simulink model "afe_inv_psm_n"  (R2026b)
settings: Solver=ode23tb  StopTime=param.sim.simlength  FixedStep=param.sim.tc  MaxStep=param.glb_time.tc
values from neighbouring files (symbols this model uses):
  param = struct()    [init_model.m]
libraries: fl_lib x30, nesl_utility x17, single_phase_transformer_lib x3, grid_following_dqctrl x2, pmsm_inverter_dqctrl x2, cstblocks_lti x2, three_phase_voltage_with_frt_emulator_mfcn x1, simple_flexible_shaft x1, permanent_magnet_synchronous_machine x1
(part 1 of 2)
settings Model: Creator=dbagn  LastModifiedBy=d.bagnara
settings SolverCC: SolverResetMethod=Robust  ZeroCrossControl=DisableAll
settings DataIOCC: DSMLogging=off  ReturnWorkspaceOutputs=off  SaveOutput=off  SaveTime=off  SignalLogging=off
settings OptimizationCC: ReuseModelBlockBuffer=off
settings SFSimCC: CustomCodeUndefinedFunction=ThrowError  DefaultCustomCodeDeterministicFunctions=All
settings SFSimCC: SimCustomHeaderCode=|
  | #include "rpi.h"
  | #include "mavgflt.h"
  | #include "mavgflt_simulink.h"
  | #include "mavgflts.h"
  | #include "mavgflts_simulink.h"
  | #include "dsmavgflt.h"
  | #include "dsmavgflt_simulink.h"
  | #include "bemf_obsv.h"
  | #include "bemf_obsv_simulink.h"
  | #include "bemf_obsv_load_est.h"
  | #include "bemf_obsv_load_est_simulink.h"
  | #include "dqvector_pi.h"
  | #include "dqvector_pi_simulink.h"
  | #include "sv_pwm_simulink.h"
  | #include "sv_pwm.h"
  | #include "first_harmonic_tracker.h"
  | #include "first_harmonic_tracker_simulink.h"
  | #include "dqpll_thyr.h"
  | #include "dqpll_thyr_simulink.h"
  | #include "dqpll_grid.h"
  | #include "dqpll_grid_simulink.h"
  | #include "linear_double_integrator_observer_simulink.h"
  | #include "linear_double_integrator_observer.h"
  | #include "sv_pwm_cm_simulink.h"
  | #include "sv_pwm_cm.h"
settings SFSimCC: SimUserIncludeDirs=|
  | include
  | src
settings SFSimCC: SimUserSources=|
  | "rpi.c"
  | "mavgflt_simulink.c"
  | "mavgflt.c"
  | "mavgflts_simulink.c"
  | "mavgflts.c"
  | "dsmavgflt_simulink.c"
  | "dsmavgflt.c"
  | "bemf_obsv_simulink.c"
  | "bemf_obsv.c"
  | "bemf_obsv_load_est_simulink.c"
  | "bemf_obsv_load_est.c"
  | "dqvector_pi.c"
  | "dqvector_pi_simulink.c"
  | "sv_pwm_simulink.c"
  | "sv_pwm.c"
  | "first_harmonic_tracker_simulink.c"
  | "first_harmonic_tracker.c"
  | "dqpll_thyr_simulink.c"
  | "dqpll_thyr.c"
  | "dqpll_grid_simulink.c"
  | "dqpll_grid.c"
  | "linear_double_integrator_observer_simulink.c"
  | "linear_double_integrator_observer.c"
  | "sv_pwm_cm_simulink.c"
  | "sv_pwm_cm.c"
settings RTWCC: DLArmComputeVersion=19.05
settings SimscapeCC: SimscapeUseEnergyAccounting=off

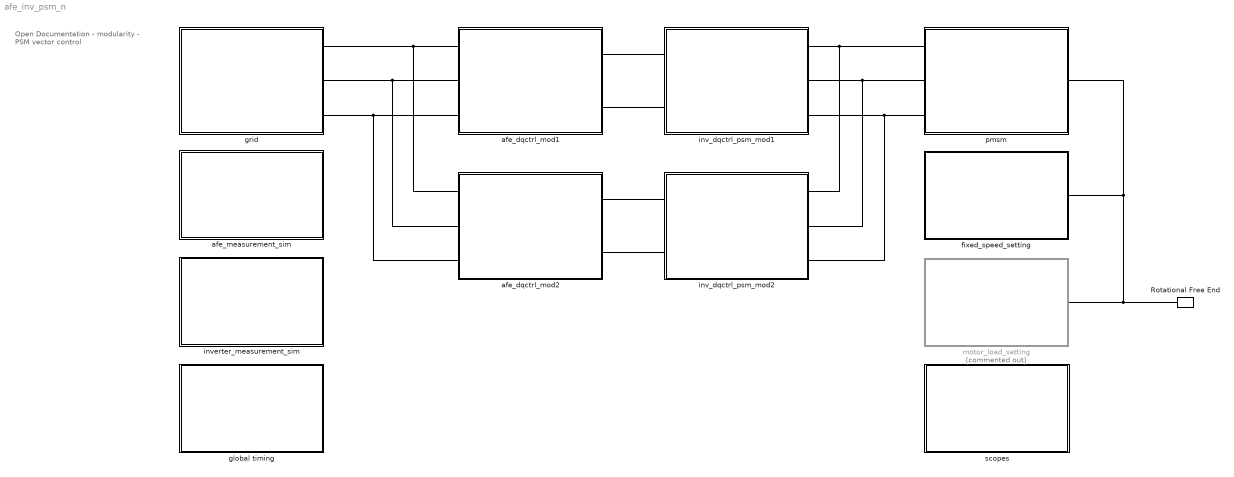
== system afe_inv_psm_n ==
  note: Open Documentation
      | - modularity
      | - PSM vector control
  Rotational Free End : fl_lib/Mechanical/Rotational Elements/Rotational Free End  w_specify=off  w_priority=None  w=0 rad/s  w_nominal_specify=off  w_nominal_value=1  w_nominal_unit=rad/s
  afe_dqctrl_mod1 : Subsystem
  afe_dqctrl_mod2 : Subsystem
  afe_measurement_sim : Subsystem
  fixed_speed_setting : Subsystem
  global timing : Subsystem
  grid : Subsystem
  inv_dqctrl_psm_mod1 : Subsystem
  inv_dqctrl_psm_mod2 : Subsystem
  inverter_measurement_sim : Subsystem
  motor_load_setting : Subsystem  Commented=on
  pmsm : Subsystem
  scopes : Subsystem
  connections:
  pmsm/RConn1 -- motor_load_setting/LConn1 -- Rotational Free End/LConn1 -- fixed_speed_setting/LConn1
  inv_dqctrl_psm_mod1/LConn1 -- afe_dqctrl_mod1/RConn1
  inv_dqctrl_psm_mod1/LConn2 -- afe_dqctrl_mod1/RConn2
  grid/RConn1 -- afe_dqctrl_mod1/LConn1 -- afe_dqctrl_mod2/LConn1
  grid/RConn2 -- afe_dqctrl_mod1/LConn2 -- afe_dqctrl_mod2/LConn2
  grid/RConn3 -- afe_dqctrl_mod1/LConn3 -- afe_dqctrl_mod2/LConn3
  inv_dqctrl_psm_mod1/RConn1 -- inv_dqctrl_psm_mod2/RConn1 -- pmsm/LConn1
  inv_dqctrl_psm_mod1/RConn2 -- inv_dqctrl_psm_mod2/RConn2 -- pmsm/LConn2
  inv_dqctrl_psm_mod1/RConn3 -- inv_dqctrl_psm_mod2/RConn3 -- pmsm/LConn3
  inv_dqctrl_psm_mod2/LConn2 -- afe_dqctrl_mod2/RConn2
  inv_dqctrl_psm_mod2/LConn1 -- afe_dqctrl_mod2/RConn1

== system afe_inv_psm_n/afe_dqctrl_mod1 ==
  grid_following_dqctrl_mod1 : grid_following_dqctrl/grid_following_dqctrl_mod1  p=param.afe_follower(1)
  ug_a : PMIOPort  Side=Left
  ug_b : PMIOPort  Port=2  Side=Left
  ug_c : PMIOPort  Port=3  Side=Left
  Udc(+) : PMIOPort  Port=4  Side=Right
  Udc(-) : PMIOPort  Port=5  Side=Right
  wires:
  [time_afe_module_1] -> grid_following_dqctrl_mod1/1
  connections:
  grid_following_dqctrl_mod1/LConn3 -- ug_c/RConn1
  grid_following_dqctrl_mod1/LConn1 -- ug_a/RConn1
  grid_following_dqctrl_mod1/RConn2 -- Udc(-)/RConn1
  grid_following_dqctrl_mod1/LConn2 -- ug_b/RConn1
  grid_following_dqctrl_mod1/RConn1 -- Udc(+)/RConn1

== system afe_inv_psm_n/afe_dqctrl_mod2 ==
  grid_following_dqctrl_mod2 : grid_following_dqctrl/grid_following_dqctrl_mod1  p=param.afe_follower(2)
  ug_a : PMIOPort  Side=Left
  ug_b : PMIOPort  Port=2  Side=Left
  ug_c : PMIOPort  Port=3  Side=Left
  Udc(+) : PMIOPort  Port=4  Side=Right
  Udc(-) : PMIOPort  Port=5  Side=Right
  wires:
  [time_afe_module_2] -> grid_following_dqctrl_mod2/1
  connections:
  grid_following_dqctrl_mod2/RConn1 -- Udc(+)/RConn1
  grid_following_dqctrl_mod2/LConn2 -- ug_b/RConn1
  grid_following_dqctrl_mod2/RConn2 -- Udc(-)/RConn1
  grid_following_dqctrl_mod2/LConn1 -- ug_a/RConn1
  grid_following_dqctrl_mod2/LConn3 -- ug_c/RConn1

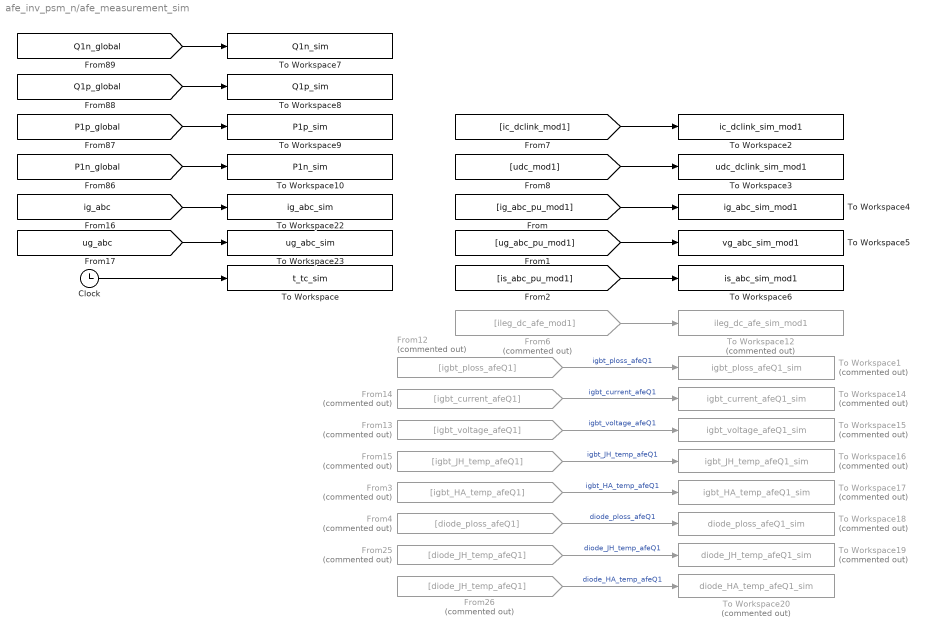
== system afe_inv_psm_n/afe_measurement_sim ==
  Clock : Clock
  From12 : From  Commented=on  GotoTag=igbt_ploss_afeQ1
  From13 : From  Commented=on  GotoTag=igbt_voltage_afeQ1
  From14 : From  Commented=on  GotoTag=igbt_current_afeQ1
  From15 : From  Commented=on  GotoTag=igbt_JH_temp_afeQ1
  From25 : From  Commented=on  GotoTag=diode_JH_temp_afeQ1
  From26 : From  Commented=on  GotoTag=diode_JH_temp_afeQ1
  From3 : From  Commented=on  GotoTag=igbt_HA_temp_afeQ1
  From4 : From  Commented=on  GotoTag=diode_ploss_afeQ1
  From6 : From  Commented=on  GotoTag=ileg_dc_afe_mod1
  To Workspace : ToWorkspace  VariableName=t_tc_sim  SampleTime=param.glb_time.tc
      settings: MaxDataPoints=param.glb_time.Nc
  To Workspace1 : ToWorkspace  Commented=on  VariableName=igbt_ploss_afeQ1_sim  SampleTime=param.glb_time.tc
      settings: MaxDataPoints=param.glb_time.Nc
  To Workspace10 : ToWorkspace  VariableName=P1n_sim  SampleTime=param.glb_time.ts_afe
      settings: MaxDataPoints=param.glb_time.Ns_afe
  To Workspace12 : ToWorkspace  Commented=on  VariableName=ileg_dc_afe_sim_mod1  SampleTime=param.glb_time.tc
      settings: MaxDataPoints=param.glb_time.Nc
  To Workspace14 : ToWorkspace  Commented=on  VariableName=igbt_current_afeQ1_sim  SampleTime=param.glb_time.tc
      settings: MaxDataPoints=param.glb_time.Nc
  To Workspace15 : ToWorkspace  Commented=on  VariableName=igbt_voltage_afeQ1_sim  SampleTime=param.glb_time.tc
      settings: MaxDataPoints=param.glb_time.Nc
  To Workspace16 : ToWorkspace  Commented=on  VariableName=igbt_JH_temp_afeQ1_sim  SampleTime=param.glb_time.tc
      settings: MaxDataPoints=param.glb_time.Nc
  To Workspace17 : ToWorkspace  Commented=on  VariableName=igbt_HA_temp_afeQ1_sim  SampleTime=param.glb_time.tc
      settings: MaxDataPoints=param.glb_time.Nc
  To Workspace18 : ToWorkspace  Commented=on  VariableName=diode_ploss_afeQ1_sim  SampleTime=param.glb_time.tc
      settings: MaxDataPoints=param.glb_time.Nc
  To Workspace19 : ToWorkspace  Commented=on  VariableName=diode_JH_temp_afeQ1_sim  SampleTime=param.glb_time.tc
      settings: MaxDataPoints=param.glb_time.Nc
  To Workspace2 : ToWorkspace  VariableName=ic_dclink_sim_mod1  SampleTime=param.glb_time.tc
      settings: MaxDataPoints=param.glb_time.Nc
  To Workspace20 : ToWorkspace  Commented=on  VariableName=diode_HA_temp_afeQ1_sim  SampleTime=param.glb_time.tc
      settings: MaxDataPoints=param.glb_time.Nc
  To Workspace22 : ToWorkspace  VariableName=ig_abc_sim  SampleTime=param.glb_time.tc
      settings: MaxDataPoints=param.glb_time.Nc
  To Workspace23 : ToWorkspace  VariableName=ug_abc_sim  SampleTime=param.glb_time.tc
      settings: MaxDataPoints=param.glb_time.Nc
  To Workspace3 : ToWorkspace  VariableName=udc_dclink_sim_mod1  SampleTime=param.glb_time.tc
      settings: MaxDataPoints=param.glb_time.Nc
  To Workspace4 : ToWorkspace  VariableName=ig_abc_sim_mod1  SampleTime=param.glb_time.tc
      settings: MaxDataPoints=param.glb_time.Nc
  To Workspace5 : ToWorkspace  VariableName=vg_abc_sim_mod1  SampleTime=param.glb_time.tc
      settings: MaxDataPoints=param.glb_time.Nc
  To Workspace6 : ToWorkspace  VariableName=is_abc_sim_mod1  SampleTime=param.glb_time.tc
      settings: MaxDataPoints=param.glb_time.Nc
  To Workspace7 : ToWorkspace  VariableName=Q1n_sim  SampleTime=param.glb_time.ts_afe
      settings: MaxDataPoints=param.glb_time.Ns_afe
  To Workspace8 : ToWorkspace  VariableName=Q1p_sim  SampleTime=param.glb_time.ts_afe
      settings: MaxDataPoints=param.glb_time.Ns_afe
  To Workspace9 : ToWorkspace  VariableName=P1p_sim  SampleTime=param.glb_time.ts_afe
      settings: MaxDataPoints=param.glb_time.Ns_afe
  wires:
  Clock/1 -> To Workspace/1
  [Q1n_global] -> To Workspace7/1
  [Q1p_global] -> To Workspace8/1
  [P1p_global] -> To Workspace9/1
  [P1n_global] -> To Workspace10/1
  [ug_abc] -> To Workspace23/1
  [ig_abc] -> To Workspace22/1
  [ug_abc_pu_mod1] -> To Workspace5/1
  [ig_abc_pu_mod1] -> To Workspace4/1
  From6/1 -> To Workspace12/1
  [udc_mod1] -> To Workspace3/1
  [ic_dclink_mod1] -> To Workspace2/1
  [is_abc_pu_mod1] -> To Workspace6/1
  From13/1 -> To Workspace15/1  "igbt_voltage_afeQ1"
  From3/1 -> To Workspace17/1  "igbt_HA_temp_afeQ1"
  From4/1 -> To Workspace18/1  "diode_ploss_afeQ1"
  From25/1 -> To Workspace19/1  "diode_JH_temp_afeQ1"
  From12/1 -> To Workspace1/1  "igbt_ploss_afeQ1"
  From26/1 -> To Workspace20/1  "diode_HA_temp_afeQ1"
  From14/1 -> To Workspace14/1  "igbt_current_afeQ1"
  From15/1 -> To Workspace16/1  "igbt_JH_temp_afeQ1"

== system afe_inv_psm_n/fixed_speed_setting ==
  Ideal Angular Velocity Source : fl_lib/Mechanical/Mechanical Sources/Ideal Angular Velocity Source
  Mechanical Rotational Reference : fl_lib/Mechanical/Rotational Elements/Mechanical Rotational Reference
  PS Step1 : fl_lib/Physical Signals/Sources/PS Step  step_time=0.025 s  initial_value=0 rpm  final_value=param.load.rpm_sim rpm
  PS Transfer Function : fl_lib/Physical Signals/Linear Operators/PS Transfer Function  transfer_function_type=foundation.enum.transfer_function_type.lag  T=0.1 s  T1=2 s  T2=1 s  reset_method=foundation.enum.IntegratorResetSpec.None  initial_condition_spec=foundation.enum.IntegratorICSpec.Internal  y0=0 rpm
  shaft : PMIOPort  Side=Left
  connections:
  Mechanical Rotational Reference/LConn1 -- Ideal Angular Velocity Source/RConn2
  PS Step1/RConn1 -- PS Transfer Function/LConn1
  PS Transfer Function/RConn1 -- Ideal Angular Velocity Source/RConn1
  Ideal Angular Velocity Source/LConn1 -- shaft/RConn1

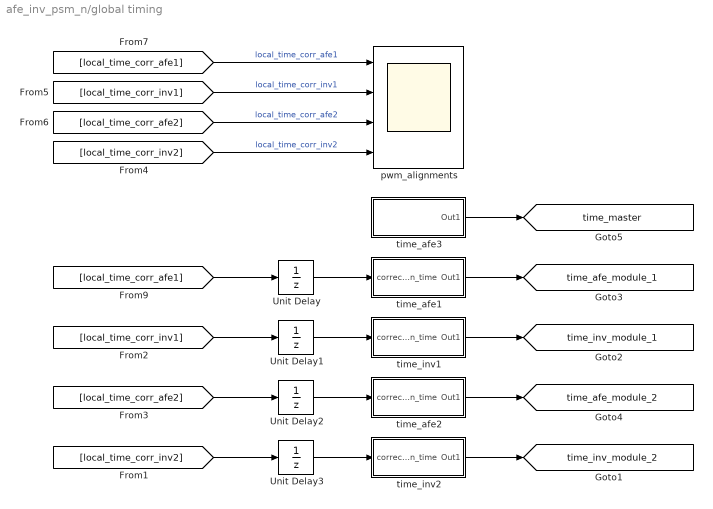
== system afe_inv_psm_n/global timing ==
  Unit Delay{,1..3} (4 alike) : UnitDelay  SampleTime=param.glb_time.tc
  pwm_alignments : Scope  NumInputPorts=4
      settings: SampleTime=param.glb_time.tc  ActiveDisplayYMinimum=-1  ActiveDisplayYMaximum=1  DataLoggingVariableName=ScopeData40
  time_afe1 : Subsystem  mask{k=param.afe.behav.time_gain_module_1}
      mask prompts: k "Time Gain"
      mask Display:
      | disp('time-gen');
      | port_label('input', 1, 'crt');
      | port_label('output', 1, 'tout');
  time_afe2 : Subsystem  mask{k=param.afe.behav.time_gain_module_2}
      mask prompts: k "Time Gain"
      mask Display:
      | disp('time-gen');
      | port_label('input', 1, 'crt');
      | port_label('output', 1, 'tout');
  time_afe3 : Subsystem  mask{k=1}
      mask prompts: k "Time Gain"
      mask Display:
      | disp('time-gen');
      | port_label('output', 1, 'tout');
  time_inv1 : Subsystem  mask{k=param.inv.behav.time_gain_module_1}
      mask prompts: k "Time Gain"
      mask Display:
      | disp('time-gen');
      | port_label('input', 1, 'crt');
      | port_label('output', 1, 'tout');
  time_inv2 : Subsystem  mask{k=param.inv.behav.time_gain_module_2}
      mask prompts: k "Time Gain"
      mask Display:
      | disp('time-gen');
      | port_label('input', 1, 'crt');
      | port_label('output', 1, 'tout');
  tag scope: time_afe_module_1=global, time_afe_module_2=global, time_inv_module_1=global, time_inv_module_2=global, time_master=global
  wires:
  time_afe1/1(Out1) -> [time_afe_module_1]
  time_inv1/1(Out1) -> [time_inv_module_1]
  time_afe3/1(Out1) -> [time_master]
  [local_time_corr_afe1] -> Unit Delay/1
  [local_time_corr_inv1] -> Unit Delay1/1
  [local_time_corr_inv2] -> Unit Delay3/1
  [local_time_corr_afe2] -> Unit Delay2/1
  time_inv2/1(Out1) -> [time_inv_module_2]
  time_afe2/1(Out1) -> [time_afe_module_2]
  Unit Delay/1 -> time_afe1/1(correction_time)
  Unit Delay1/1 -> time_inv1/1(correction_time)
  Unit Delay2/1 -> time_afe2/1(correction_time)
  Unit Delay3/1 -> time_inv2/1(correction_time)
  [local_time_corr_afe1] -> pwm_alignments/1  "local_time_corr_afe1"
  [local_time_corr_inv1] -> pwm_alignments/2  "local_time_corr_inv1"
  [local_time_corr_afe2] -> pwm_alignments/3  "local_time_corr_afe2"
  [local_time_corr_inv2] -> pwm_alignments/4  "local_time_corr_inv2"

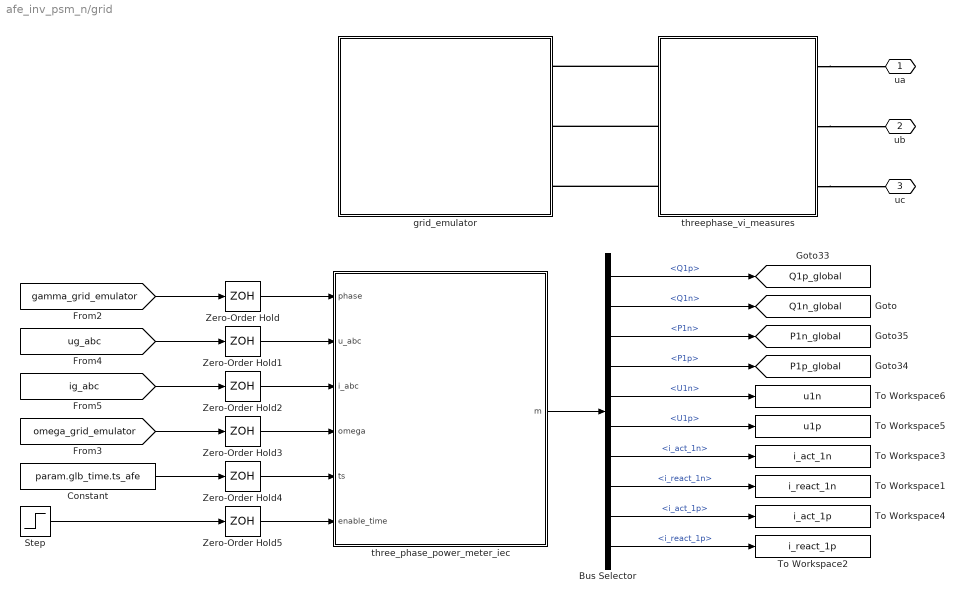
== system afe_inv_psm_n/grid ==
  Bus Selector : BusSelector  OutputSignals=Q1p,Q1n,P1n,P1p,U1n,U1p,i_act_1n,i_react_1n,i_act_1p,i_react_1p
  Constant : Constant  Value=param.glb_time.ts_afe
  Step : Step  Time=0.025  InitialValue=1  FinalValue=0  SampleTime=0
  To Workspace1 : ToWorkspace  VariableName=i_react_1n  SampleTime=param.glb_time.ts_afe
      settings: MaxDataPoints=param.glb_time.Ns_afe
  To Workspace2 : ToWorkspace  VariableName=i_react_1p  SampleTime=param.glb_time.ts_afe
      settings: MaxDataPoints=param.glb_time.Ns_afe
  To Workspace3 : ToWorkspace  VariableName=i_act_1n  SampleTime=param.glb_time.ts_afe
      settings: MaxDataPoints=param.glb_time.Ns_afe
  To Workspace4 : ToWorkspace  VariableName=i_act_1p  SampleTime=param.glb_time.ts_afe
      settings: MaxDataPoints=param.glb_time.Ns_afe
  To Workspace5 : ToWorkspace  VariableName=u1p  SampleTime=param.glb_time.ts_afe
      settings: MaxDataPoints=param.glb_time.Ns_afe
  To Workspace6 : ToWorkspace  VariableName=u1n  SampleTime=param.glb_time.ts_afe
      settings: MaxDataPoints=param.glb_time.Ns_afe
  Zero-Order Hold{,1..5} (6 alike) : ZeroOrderHold  SampleTime=param.glb_time.ts_afe
  grid_emulator : Subsystem
  three_phase_power_meter_iec : MATLAB Function  TreatAsAtomicUnit=on  SystemSampleTime=param.glb_time.ts_afe
  threephase_vi_measures : Subsystem
  ua : PMIOPort  Side=Right
  ub : PMIOPort  Port=2  Side=Right
  uc : PMIOPort  Port=3  Side=Right
  tag scope: P1n_global=global, P1p_global=global, Q1n_global=global, Q1p_global=global
  wires:
  three_phase_power_meter_iec/1(m) -> Bus Selector/1
  Bus Selector/1 -> [Q1p_global]  "<Q1p>"
  Bus Selector/2 -> [Q1n_global]  "<Q1n>"
  Bus Selector/3 -> [P1n_global]  "<P1n>"
  Bus Selector/4 -> [P1p_global]  "<P1p>"
  Bus Selector/5 -> To Workspace6/1  "<U1n>"
  Bus Selector/6 -> To Workspace5/1  "<U1p>"
  Bus Selector/7 -> To Workspace3/1  "<i_act_1n>"
  Bus Selector/8 -> To Workspace1/1  "<i_react_1n>"
  Bus Selector/9 -> To Workspace4/1  "<i_act_1p>"
  Bus Selector/10 -> To Workspace2/1  "<i_react_1p>"
  Zero-Order Hold4/1 -> three_phase_power_meter_iec/5(ts)
  Step/1 -> Zero-Order Hold5/1
  [gamma_grid_emulator] -> Zero-Order Hold/1
  [ug_abc] -> Zero-Order Hold1/1
  Zero-Order Hold1/1 -> three_phase_power_meter_iec/2(u_abc)
  [ig_abc] -> Zero-Order Hold2/1
  [omega_grid_emulator] -> Zero-Order Hold3/1
  Constant/1 -> Zero-Order Hold4/1
  Zero-Order Hold3/1 -> three_phase_power_meter_iec/4(omega)
  Zero-Order Hold/1 -> three_phase_power_meter_iec/1(phase)
  Zero-Order Hold5/1 -> three_phase_power_meter_iec/6(enable_time)
  Zero-Order Hold2/1 -> three_phase_power_meter_iec/3(i_abc)
  connections:
  threephase_vi_measures/LConn3 -- grid_emulator/RConn3
  threephase_vi_measures/LConn1 -- grid_emulator/RConn1
  threephase_vi_measures/RConn2 -- ub/RConn1
  threephase_vi_measures/LConn2 -- grid_emulator/RConn2
  threephase_vi_measures/RConn1 -- ua/RConn1
  threephase_vi_measures/RConn3 -- uc/RConn1

== system afe_inv_psm_n/inv_dqctrl_psm_mod1 ==
  Bus Creator : BusCreator  Inputs=2
  Constant : Constant
  Step : Step  Time=0.125  SampleTime=0
  pmsm_inverter_dqctrl_mod1 : pmsm_inverter_dqctrl/pmsm_inverter_dqctrl_mod1  p=param.inv_mod(1)
  Udc(+) : PMIOPort  Side=Left
  Udc(-) : PMIOPort  Port=2  Side=Left
  u : PMIOPort  Port=3  Side=Right
  v : PMIOPort  Port=4  Side=Right
  w : PMIOPort  Port=5  Side=Right
  wires:
  [time_inv_module_1] -> pmsm_inverter_dqctrl_mod1/1
  [theta_elec_psm] -> pmsm_inverter_dqctrl_mod1/3
  Step/1 -> Bus Creator/1  "enable"
  Constant/1 -> Bus Creator/2  "mode"
  Bus Creator/1 -> pmsm_inverter_dqctrl_mod1/2
  connections:
  pmsm_inverter_dqctrl_mod1/LConn1 -- Udc(+)/RConn1
  pmsm_inverter_dqctrl_mod1/RConn2 -- v/RConn1
  pmsm_inverter_dqctrl_mod1/RConn1 -- u/RConn1
  pmsm_inverter_dqctrl_mod1/LConn2 -- Udc(-)/RConn1
  pmsm_inverter_dqctrl_mod1/RConn3 -- w/RConn1

== system afe_inv_psm_n/inv_dqctrl_psm_mod2 ==
  Bus Creator : BusCreator  Inputs=2
  Constant : Constant
  Step : Step  Time=0.125  SampleTime=0
  pmsm_inverter_dqctrl_mod2 : pmsm_inverter_dqctrl/pmsm_inverter_dqctrl_mod1  p=param.inv_mod(2)
  Udc(+) : PMIOPort  Side=Left
  Udc(-) : PMIOPort  Port=2  Side=Left
  u : PMIOPort  Port=3  Side=Right
  v : PMIOPort  Port=4  Side=Right
  w : PMIOPort  Port=5  Side=Right
  wires:
  [time_inv_module_2] -> pmsm_inverter_dqctrl_mod2/1
  [theta_elec_psm] -> pmsm_inverter_dqctrl_mod2/3
  Bus Creator/1 -> pmsm_inverter_dqctrl_mod2/2
  Step/1 -> Bus Creator/1  "enable"
  Constant/1 -> Bus Creator/2  "mode"
  connections:
  pmsm_inverter_dqctrl_mod2/RConn3 -- w/RConn1
  pmsm_inverter_dqctrl_mod2/LConn2 -- Udc(-)/RConn1
  pmsm_inverter_dqctrl_mod2/RConn1 -- u/RConn1
  pmsm_inverter_dqctrl_mod2/RConn2 -- v/RConn1
  pmsm_inverter_dqctrl_mod2/LConn1 -- Udc(+)/RConn1

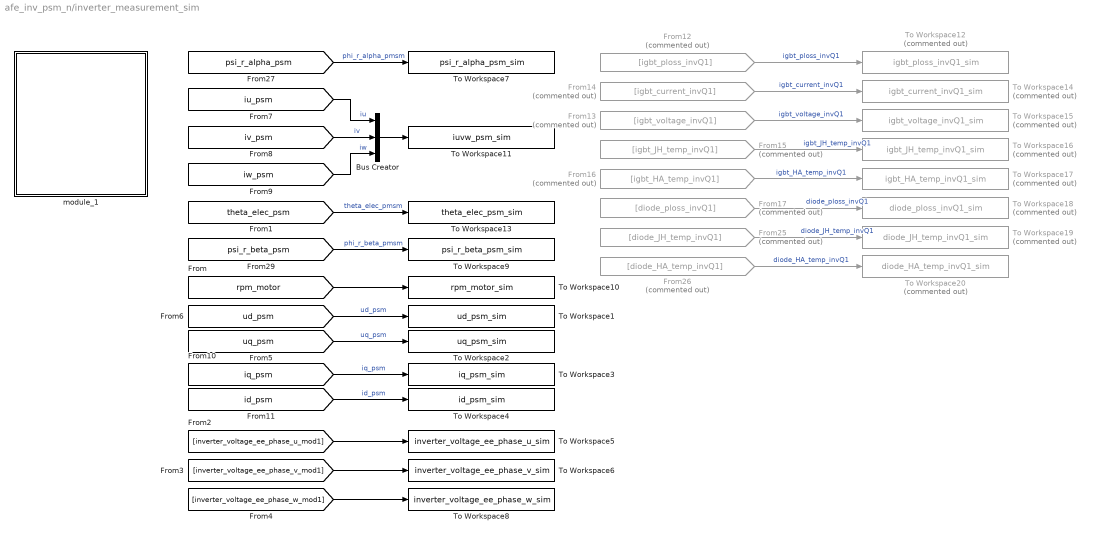
== system afe_inv_psm_n/inverter_measurement_sim ==
  Bus Creator : BusCreator  Inputs=3
  From12 : From  Commented=on  GotoTag=igbt_ploss_invQ1
  From13 : From  Commented=on  GotoTag=igbt_voltage_invQ1
  From14 : From  Commented=on  GotoTag=igbt_current_invQ1
  From15 : From  Commented=on  GotoTag=igbt_JH_temp_invQ1
  From16 : From  Commented=on  GotoTag=igbt_HA_temp_invQ1
  From17 : From  Commented=on  GotoTag=diode_ploss_invQ1
  From25 : From  Commented=on  GotoTag=diode_JH_temp_invQ1
  From26 : From  Commented=on  GotoTag=diode_HA_temp_invQ1
  To Workspace1 : ToWorkspace  VariableName=ud_psm_sim  SampleTime=param.glb_time.tc
      settings: MaxDataPoints=param.glb_time.Nc
  To Workspace10 : ToWorkspace  VariableName=rpm_motor_sim  SampleTime=param.glb_time.tc
      settings: MaxDataPoints=param.glb_time.Nc
  To Workspace11 : ToWorkspace  VariableName=iuvw_psm_sim  SampleTime=param.glb_time.tc
      settings: MaxDataPoints=param.glb_time.Nc
  To Workspace12 : ToWorkspace  Commented=on  VariableName=igbt_ploss_invQ1_sim  SampleTime=param.glb_time.tc
      settings: MaxDataPoints=param.glb_time.Nc
  To Workspace13 : ToWorkspace  VariableName=theta_elec_psm_sim  SampleTime=param.glb_time.tc
      settings: MaxDataPoints=param.glb_time.Nc
  To Workspace14 : ToWorkspace  Commented=on  VariableName=igbt_current_invQ1_sim  SampleTime=param.glb_time.tc
      settings: MaxDataPoints=param.glb_time.Nc
  To Workspace15 : ToWorkspace  Commented=on  VariableName=igbt_voltage_invQ1_sim  SampleTime=param.glb_time.tc
      settings: MaxDataPoints=param.glb_time.Nc
  To Workspace16 : ToWorkspace  Commented=on  VariableName=igbt_JH_temp_invQ1_sim  SampleTime=param.glb_time.tc
      settings: MaxDataPoints=param.glb_time.Nc
  To Workspace17 : ToWorkspace  Commented=on  VariableName=igbt_HA_temp_invQ1_sim  SampleTime=param.glb_time.tc
      settings: MaxDataPoints=param.glb_time.Nc
  To Workspace18 : ToWorkspace  Commented=on  VariableName=diode_ploss_invQ1_sim  SampleTime=param.glb_time.tc
      settings: MaxDataPoints=param.glb_time.Nc
  To Workspace19 : ToWorkspace  Commented=on  VariableName=diode_JH_temp_invQ1_sim  SampleTime=param.glb_time.tc
      settings: MaxDataPoints=param.glb_time.Nc
  To Workspace2 : ToWorkspace  VariableName=uq_psm_sim  SampleTime=param.glb_time.tc
      settings: MaxDataPoints=param.glb_time.Nc
  To Workspace20 : ToWorkspace  Commented=on  VariableName=diode_HA_temp_invQ1_sim  SampleTime=param.glb_time.tc
      settings: MaxDataPoints=param.glb_time.Nc
  To Workspace3 : ToWorkspace  VariableName=iq_psm_sim  SampleTime=param.glb_time.tc
      settings: MaxDataPoints=param.glb_time.Nc
  To Workspace4 : ToWorkspace  VariableName=id_psm_sim  SampleTime=param.glb_time.tc
      settings: MaxDataPoints=param.glb_time.Nc
  To Workspace5 : ToWorkspace  VariableName=inverter_voltage_ee_phase_u_sim  SampleTime=param.glb_time.tc
      settings: MaxDataPoints=param.glb_time.Nc
  To Workspace6 : ToWorkspace  VariableName=inverter_voltage_ee_phase_v_sim  SampleTime=param.glb_time.tc
      settings: MaxDataPoints=param.glb_time.Nc
  To Workspace7 : ToWorkspace  VariableName=psi_r_alpha_psm_sim  SampleTime=param.glb_time.tc
      settings: MaxDataPoints=param.glb_time.Nc
  To Workspace8 : ToWorkspace  VariableName=inverter_voltage_ee_phase_w_sim  SampleTime=param.glb_time.tc
      settings: MaxDataPoints=param.glb_time.Nc
  To Workspace9 : ToWorkspace  VariableName=psi_r_beta_psm_sim  SampleTime=param.glb_time.tc
      settings: MaxDataPoints=param.glb_time.Nc
  module_1 : Subsystem
  wires:
  [psi_r_alpha_psm] -> To Workspace7/1  "phi_r_alpha_pmsm"
  [psi_r_beta_psm] -> To Workspace9/1  "phi_r_beta_pmsm"
  [rpm_motor] -> To Workspace10/1
  [iv_psm] -> Bus Creator/2  "iv"
  [iw_psm] -> Bus Creator/3  "iw"
  [iu_psm] -> Bus Creator/1  "iu"
  Bus Creator/1 -> To Workspace11/1
  [theta_elec_psm] -> To Workspace13/1  "theta_elec_pmsm"
  [ud_psm] -> To Workspace1/1  "ud_psm"
  [uq_psm] -> To Workspace2/1  "uq_psm"
  [iq_psm] -> To Workspace3/1  "iq_psm"
  [id_psm] -> To Workspace4/1  "id_psm"
  [inverter_voltage_ee_phase_u_mod1] -> To Workspace5/1
  [inverter_voltage_ee_phase_v_mod1] -> To Workspace6/1
  [inverter_voltage_ee_phase_w_mod1] -> To Workspace8/1
  From26/1 -> To Workspace20/1  "diode_HA_temp_invQ1"
  From14/1 -> To Workspace14/1  "igbt_current_invQ1"
  From17/1 -> To Workspace18/1  "diode_ploss_invQ1"
  From25/1 -> To Workspace19/1  "diode_JH_temp_invQ1"
  From16/1 -> To Workspace17/1  "igbt_HA_temp_invQ1"
  From12/1 -> To Workspace12/1  "igbt_ploss_invQ1"
  From13/1 -> To Workspace15/1  "igbt_voltage_invQ1"
  From15/1 -> To Workspace16/1  "igbt_JH_temp_invQ1"

== system afe_inv_psm_n/motor_load_setting ==
  Ideal Torque Source : fl_lib/Mechanical/Mechanical Sources/Ideal Torque Source
  Inertia : fl_lib/Mechanical/Rotational Elements/Inertia  inertia=param.load.external_load_inertia kg*m^2  num_ports=foundation.enum.numPorts2.one  w_specify=off  w_priority=High  w=0 rad/s  w_nominal_specify=off  w_nominal_value=1  w_nominal_unit=rad/s  t_specify=off  t_priority=None  t=0 N*m  t_nominal_specify=off  t_nominal_value=1  t_nominal_unit=N*m
  Mechanical Rotational Reference : fl_lib/Mechanical/Rotational Elements/Mechanical Rotational Reference
  PS Step : fl_lib/Physical Signals/Sources/PS Step  step_time=param.sim.load_step_time s  initial_value=1 N*m  final_value=1 N*m
  PS Transfer Function : fl_lib/Physical Signals/Linear Operators/PS Transfer Function  transfer_function_type=foundation.enum.transfer_function_type.lag  T=1 s  T1=2 s  T2=1 s  reset_method=foundation.enum.IntegratorResetSpec.None  initial_condition_spec=foundation.enum.IntegratorICSpec.Internal  y0=0 N*m
  flexible_shaft : simple_flexible_shaft/flexible_shaft  b1=1  b2=1  J1=1  J2=1  b_displacement=1  k_displacement=1e5
  shaft : PMIOPort  Side=Left
  connections:
  Ideal Torque Source/LConn1 -- flexible_shaft/RConn1 -- Inertia/LConn1
  Ideal Torque Source/RConn2 -- Mechanical Rotational Reference/LConn1
  PS Transfer Function/RConn1 -- Ideal Torque Source/RConn1
  PS Step/RConn1 -- PS Transfer Function/LConn1
  flexible_shaft/LConn1 -- shaft/RConn1

== system afe_inv_psm_n/pmsm ==
  Bus Selector1 : BusSelector  OutputSignals=omega_mech (rpm)
  Constant : Constant  Value=param.psm.machine.psi_m
  Simulink-PS Converter3 : nesl_utility/Simulink-PS Converter  PhysicalDomain=network_engine_domain  SubClassName=ps_input  LeftPortType=input  RightPortType=output  PseudoPeriodic=off  Frequencies=[]  NoiseDistribution=none  NoiseParameters=[]  Unit=V*s  AffineConversion=on  FilteringAndDerivatives=provide  SimscapeFilterOrder=1  InputFilterTimeConstant=0.001  UdotUserProvided=0
  synchronous_motor : Subsystem
  u : PMIOPort  Side=Left
  v : PMIOPort  Port=2  Side=Left
  w : PMIOPort  Port=3  Side=Left
  shaft : PMIOPort  Port=4  Side=Right
  tag scope: rpm_motor=global
  wires:
  synchronous_motor/1(motor_data) -> Bus Selector1/1
  Bus Selector1/1 -> [rpm_motor]  "<omega_mech (rpm)>"
  Constant/1 -> Simulink-PS Converter3/1
  connections:
  synchronous_motor/LConn1 -- u/RConn1
  Simulink-PS Converter3/RConn1 -- synchronous_motor/LConn4
  synchronous_motor/LConn3 -- w/RConn1
  synchronous_motor/LConn2 -- v/RConn1
  shaft/RConn1 -- synchronous_motor/RConn1

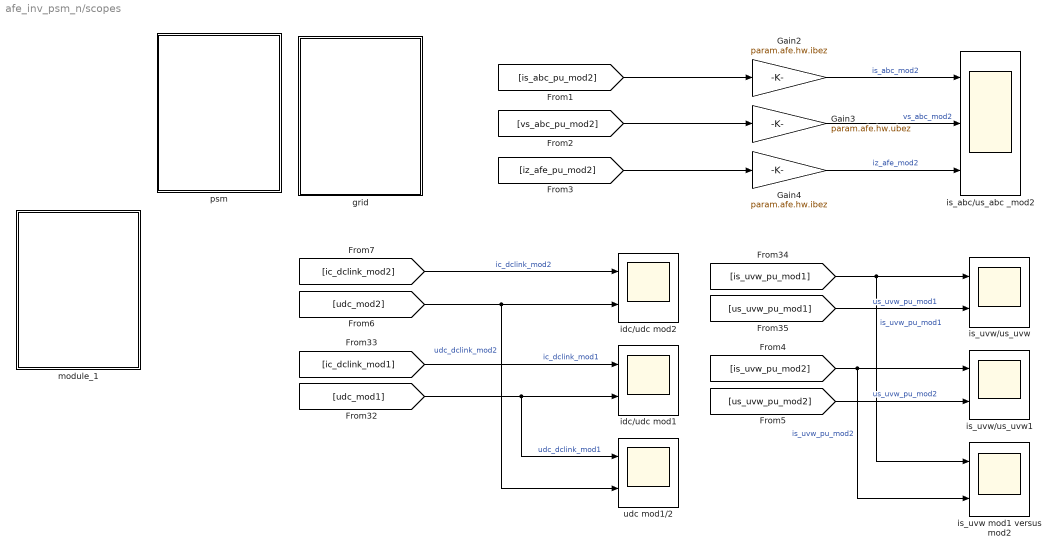
== system afe_inv_psm_n/scopes ==
  Gain2 : Gain  Gain=param.afe.hw.ibez
  Gain3 : Gain  Gain=param.afe.hw.ubez
  Gain4 : Gain  Gain=param.afe.hw.ibez
  grid : Subsystem
  idc/udc mod1 : Scope  NumInputPorts=2
      settings: SampleTime=param.glb_time.tc  ActiveDisplayYMinimum=-1001.6327830736943  ActiveDisplayYMaximum=1377.7743036043239  DataLoggingVariableName=ScopeData23
  idc/udc mod2 : Scope  NumInputPorts=2
      settings: SampleTime=param.glb_time.tc  ActiveDisplayYMinimum=-620.47896735519328  ActiveDisplayYMaximum=526.61048231653035  DataLoggingVariableName=ScopeData38
  is_abc/us_abc _mod2 : Scope  NumInputPorts=3
      settings: SampleTime=param.glb_time.tc  ActiveDisplayYMinimum=-1839.9222668184293  ActiveDisplayYMaximum=1737.4961695685106  DataLoggingVariableName=ScopeData35
  is_uvw mod1 versus mod2 : Scope  NumInputPorts=2
      settings: SampleTime=param.glb_time.tc  ActiveDisplayYMinimum=-1.1647857894412872  ActiveDisplayYMaximum=1.2042218113148759  DataLoggingVariableName=ScopeData36
  is_uvw/us_uvw : Scope  NumInputPorts=2
      settings: SampleTime=param.glb_time.tc  ActiveDisplayYMinimum=-1.2325569675038333  ActiveDisplayYMaximum=1.2339333833020862  DataLoggingVariableName=ScopeData25
  is_uvw/us_uvw1 : Scope  NumInputPorts=2
      settings: SampleTime=param.glb_time.tc  ActiveDisplayYMinimum=-1.2325569675038333  ActiveDisplayYMaximum=1.2339333833020862  DataLoggingVariableName=ScopeData37
  module_1 : Subsystem
  psm : Subsystem
  udc mod1/2 : Scope  NumInputPorts=2
      settings: SampleTime=param.glb_time.tc  ActiveDisplayYMinimum=-160.95210355128603  ActiveDisplayYMaximum=1430.9962376518129  DataLoggingVariableName=ScopeData39
  wires:
  [ic_dclink_mod1] -> idc/udc mod1/1  "ic_dclink_mod1"
  [udc_mod1] -> udc mod1/2/1, idc/udc mod1/2  "udc_dclink_mod1"
  [is_uvw_pu_mod1] -> is_uvw mod1 versus mod2/1, is_uvw/us_uvw/1  "is_uvw_pu_mod1"
  [us_uvw_pu_mod1] -> is_uvw/us_uvw/2  "us_uvw_pu_mod1"
  Gain4/1 -> is_abc/us_abc _mod2/3  "iz_afe_mod2"
  Gain3/1 -> is_abc/us_abc _mod2/2  "vs_abc_mod2"
  [iz_afe_pu_mod2] -> Gain4/1
  [vs_abc_pu_mod2] -> Gain3/1
  [is_abc_pu_mod2] -> Gain2/1
  Gain2/1 -> is_abc/us_abc _mod2/1  "is_abc_mod2"
  [us_uvw_pu_mod2] -> is_uvw/us_uvw1/2  "us_uvw_pu_mod2"
  [is_uvw_pu_mod2] -> is_uvw mod1 versus mod2/2, is_uvw/us_uvw1/1  "is_uvw_pu_mod2"
  [udc_mod2] -> udc mod1/2/2, idc/udc mod2/2  "udc_dclink_mod2"
  [ic_dclink_mod2] -> idc/udc mod2/1  "ic_dclink_mod2"

== system afe_inv_psm_n/global timing/time_afe1 ==
  correction_time : Inport
  Constant : Constant
  Gain : Gain  Gain=k
  Product : Product
  Sum : Sum  Inputs=|++
  time_1 : Clock
  Out1 : Outport
  wires:
  time_1/1 -> Gain/1
  Gain/1 -> Product/1
  Product/1 -> Out1/1
  correction_time/1 -> Sum/1
  Sum/1 -> Product/2
  Constant/1 -> Sum/2

== system afe_inv_psm_n/global timing/time_afe2 ==
  correction_time : Inport
  Constant : Constant
  Gain : Gain  Gain=k
  Product : Product
  Sum : Sum  Inputs=|++
  time_1 : Clock
  Out1 : Outport
  wires:
  Constant/1 -> Sum/2
  Sum/1 -> Product/2
  correction_time/1 -> Sum/1
  Product/1 -> Out1/1
  Gain/1 -> Product/1
  time_1/1 -> Gain/1

== system afe_inv_psm_n/global timing/time_afe3 ==
  Gain : Gain  Gain=k
  time_1 : Clock
  Out1 : Outport
  wires:
  Gain/1 -> Out1/1
  time_1/1 -> Gain/1

== system afe_inv_psm_n/global timing/time_inv1 ==
  correction_time : Inport
  Constant : Constant
  Gain : Gain  Gain=k
  Product : Product
  Sum : Sum  Inputs=|++
  time_1 : Clock
  Out1 : Outport
  wires:
  time_1/1 -> Gain/1
  Gain/1 -> Product/1
  Product/1 -> Out1/1
  correction_time/1 -> Sum/1
  Constant/1 -> Sum/2
  Sum/1 -> Product/2

== system afe_inv_psm_n/global timing/time_inv2 ==
  correction_time : Inport
  Constant : Constant
  Gain : Gain  Gain=k
  Product : Product
  Sum : Sum  Inputs=|++
  time_1 : Clock
  Out1 : Outport
  wires:
  Sum/1 -> Product/2
  Constant/1 -> Sum/2
  correction_time/1 -> Sum/1
  Product/1 -> Out1/1
  Gain/1 -> Product/1
  time_1/1 -> Gain/1

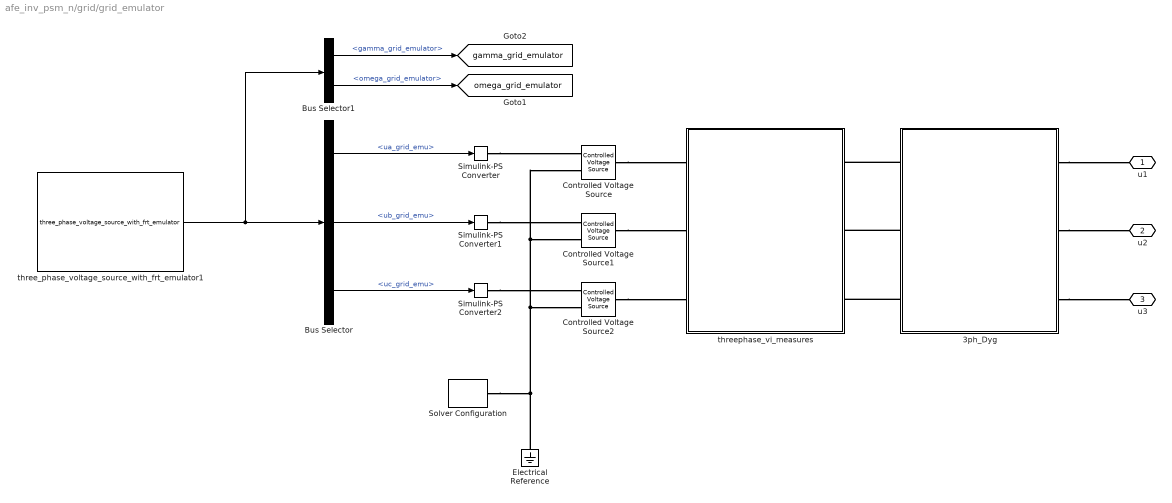
== system afe_inv_psm_n/grid/grid_emulator ==
  3ph_Dyg : Subsystem
  Bus Selector : BusSelector  OutputSignals=ua_grid_emu,ub_grid_emu,uc_grid_emu
  Bus Selector1 : BusSelector  OutputSignals=gamma_grid_emulator,omega_grid_emulator
  Controlled Voltage Source : fl_lib/Electrical/Electrical Sources/Controlled Voltage Source
  Controlled Voltage Source1 : fl_lib/Electrical/Electrical Sources/Controlled Voltage Source
  Controlled Voltage Source2 : fl_lib/Electrical/Electrical Sources/Controlled Voltage Source
  Electrical Reference : fl_lib/Electrical/Electrical Elements/Electrical Reference
  Simulink-PS Converter : nesl_utility/Simulink-PS Converter  PhysicalDomain=network_engine_domain  SubClassName=ps_input  LeftPortType=input  RightPortType=output  PseudoPeriodic=off  Frequencies=[]  NoiseDistribution=none  NoiseParameters=[]  Unit=V  AffineConversion=on  FilteringAndDerivatives=provide  SimscapeFilterOrder=1  InputFilterTimeConstant=0.001  UdotUserProvided=0
  Simulink-PS Converter1 : nesl_utility/Simulink-PS Converter  PhysicalDomain=network_engine_domain  SubClassName=ps_input  LeftPortType=input  RightPortType=output  PseudoPeriodic=off  Frequencies=[]  NoiseDistribution=none  NoiseParameters=[]  Unit=V  AffineConversion=on  FilteringAndDerivatives=provide  SimscapeFilterOrder=1  InputFilterTimeConstant=0.001  UdotUserProvided=0
  Simulink-PS Converter2 : nesl_utility/Simulink-PS Converter  PhysicalDomain=network_engine_domain  SubClassName=ps_input  LeftPortType=input  RightPortType=output  PseudoPeriodic=off  Frequencies=[]  NoiseDistribution=none  NoiseParameters=[]  Unit=V  AffineConversion=on  FilteringAndDerivatives=provide  SimscapeFilterOrder=1  InputFilterTimeConstant=0.001  UdotUserProvided=0
  Solver Configuration : nesl_utility/Solver Configuration  PhysicalDomain=network_engine_domain  SubClassName=solver  LeftPortType=input  RightPortType=generic  Tones=[]  Harmonics=[]  SimulateNoise=off  Profile=off  UseLocalSampling=off  EnableSwitchedLinearOptims=on  FrequencyDomain=off  UseCCode=off  RelTol=0.001  AbsTol=0.001  MinStep=1e-09  ToWorkspace=off  RevertToSquareIcSolve=off  NumHomotopyIterations=100  PhasorMode=off  PhasorModeNumHarmonics=1  ConsistencySolver=NEWTON_FTOL  CanonicalOrdering=UNORDERED  OptimizeIntermediates=UNOPTIMIZED  MulticoreSolverChoice=BACKWARD_EULER  IndexReductionMethod=DerivativeReplacement  DoDC=on  ResidualTolerance=1e-09  ConsistencyTolSource=GLOBAL  ConsistencyAbsTol=0.001  ConsistencyRelTol=0.001  ConsistencyTolFactor=0.001  UseLocalSolver=on  LocalSolverChoice=NE_BACKWARD_EULER_ADVANCER  ResolveIndetEquations=on  FunctionEvalNumThread=1  LocalSolverSampleTime=param.glb_time.tc  DoFixedCost=on  MaxNonlinIter=param.sim.nonlinear_iterations  MaxModeIter=2  ComputeImpulses=off  ImpulseIterations=2  LinearAlgebra=auto  LinearAlgebraNumThread=0  EquationFormulation=NE_TIME_EF  DelaysMemoryBudget=1024  AutomaticFiltering=on  FilteringTimeConstant=0.001  PartitionStorageMethod=AS_NEEDED  PartitionMemoryBudget=1024  PartitionMethod=BALANCED  MultibodyUseLocalSolver=off  MultibodyLocalSolverChoice=ODE1  MultibodyLocalSolverSampleTime=0.001
  three_phase_voltage_source_with_frt_emulator1 : three_phase_voltage_with_frt_emulator_mfcn/three_phase_voltage_source_with_frt_emulator  nominal_frequency_m=param.grid.emu.fgrid_nom  nominal_voltage_m=param.grid.emu.us_secondary_nom  Vemu_ref_norm_m=param.grid.emu.Vemu_ref_norm  vp_xi_pu_m=param.grid.emu.up_xi_pu_ref  vp_eta_pu_m=param.grid.emu.up_eta_pu_ref  vn_xi_pu_m=param.grid.emu.un_xi_pu_ref  vn_eta_pu_m=param.grid.emu.un_eta_pu_ref  Am=param.grid.emu.sof_50Hz.ss_c.A  Bm=param.grid.emu.sof_50Hz.ss_c.B  Cm=param.grid.emu.sof_50Hz.ss_c.C  enable_frt_1_m=param.grid.frt.enable_frt_1  enable_frt_2_m=param.grid.frt.enable_frt_2  start_time_LVRT_m=param.grid.frt.start_time_LVRT  end_time_LVRT_m=param.grid.frt.end_time_LVRT  deepPOSxi_m=param.grid.frt.deepPOSxi  deepPOSeta_m=param.grid.frt.deepPOSeta  deepNEGxi_m=param.grid.frt.deepNEGxi  deepNEGeta_m=param.grid.frt.deepNEGeta  Amplitude_U_m=param.grid.frt.Amplitude_U  Amplitude_V_m=param.grid.frt.Amplitude_V  Amplitude_W_m=param.grid.frt.Amplitude_W  t_ramp_m=param.grid.frt.t_ramp  Phase_shift_m=param.grid.frt.Phase_shift
  threephase_vi_measures : Subsystem
  u1 : PMIOPort  Side=Right
  u2 : PMIOPort  Port=2  Side=Right
  u3 : PMIOPort  Port=3  Side=Right
  tag scope: gamma_grid_emulator=global, omega_grid_emulator=global
  wires:
  Bus Selector1/2 -> [omega_grid_emulator]  "<omega_grid_emulator>"
  Bus Selector1/1 -> [gamma_grid_emulator]  "<gamma_grid_emulator>"
  Bus Selector/2 -> Simulink-PS Converter1/1  "<ub_grid_emu>"
  Bus Selector/3 -> Simulink-PS Converter2/1  "<uc_grid_emu>"
  three_phase_voltage_source_with_frt_emulator1/1 -> Bus Selector1/1, Bus Selector/1
  Bus Selector/1 -> Simulink-PS Converter/1  "<ua_grid_emu>"
  connections:
  Simulink-PS Converter/RConn1 -- Controlled Voltage Source/RConn1
  Simulink-PS Converter1/RConn1 -- Controlled Voltage Source1/RConn1
  Simulink-PS Converter2/RConn1 -- Controlled Voltage Source2/RConn1
  Electrical Reference/LConn1 -- Controlled Voltage Source/RConn2 -- Controlled Voltage Source1/RConn2 -- Controlled Voltage Source2/RConn2 -- Solver Configuration/RConn1
  3ph_Dyg/RConn1 -- u1/RConn1
  3ph_Dyg/RConn2 -- u2/RConn1
  3ph_Dyg/RConn3 -- u3/RConn1
  3ph_Dyg/LConn1 -- threephase_vi_measures/RConn1
  3ph_Dyg/LConn2 -- threephase_vi_measures/RConn2
  3ph_Dyg/LConn3 -- threephase_vi_measures/RConn3
  Controlled Voltage Source/LConn1 -- threephase_vi_measures/LConn1
  Controlled Voltage Source1/LConn1 -- threephase_vi_measures/LConn2
  Controlled Voltage Source2/LConn1 -- threephase_vi_measures/LConn3

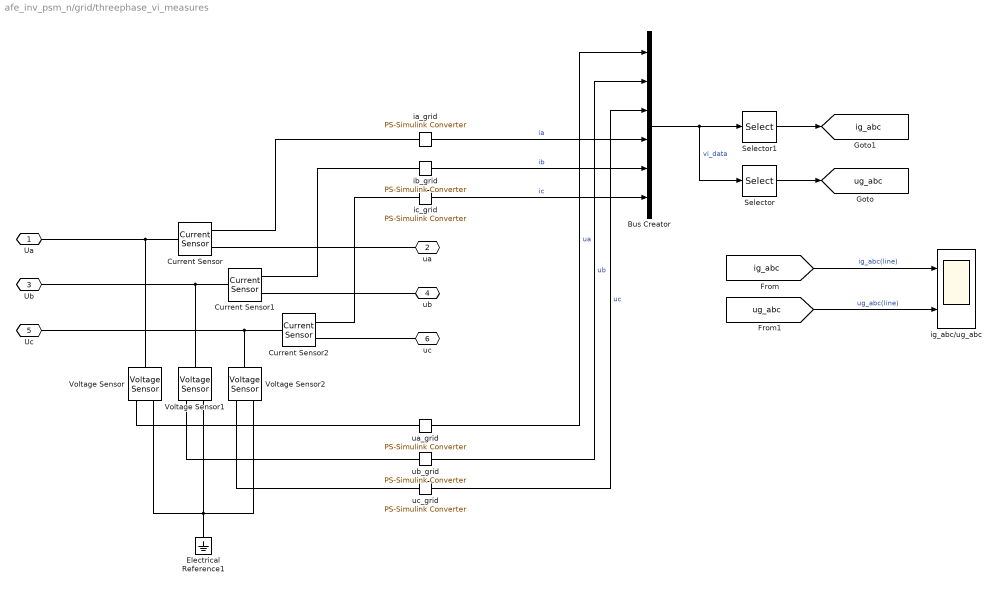
== system afe_inv_psm_n/grid/threephase_vi_measures ==
  Bus Creator : BusCreator  Inputs=6
  Current Sensor : fl_lib/Electrical/Electrical Sensors/Current Sensor
  Current Sensor1 : fl_lib/Electrical/Electrical Sensors/Current Sensor
  Current Sensor2 : fl_lib/Electrical/Electrical Sensors/Current Sensor
  Electrical Reference1 : fl_lib/Electrical/Electrical Elements/Electrical Reference
  Selector : Selector  InputPortWidth=6  IndexOptions=Index vector (dialog)  Indices=[1 2 3]  OutputSizes=1  RuntimeRangeChecks=off
  Selector1 : Selector  InputPortWidth=6  IndexOptions=Index vector (dialog)  Indices=[4 5 6]  OutputSizes=1  RuntimeRangeChecks=off
  Voltage Sensor : fl_lib/Electrical/Electrical Sensors/Voltage Sensor
  Voltage Sensor1 : fl_lib/Electrical/Electrical Sensors/Voltage Sensor
  Voltage Sensor2 : fl_lib/Electrical/Electrical Sensors/Voltage Sensor
  ia_grid : nesl_utility/PS-Simulink Converter  PhysicalDomain=network_engine_domain  SubClassName=ps_output  LeftPortType=input  RightPortType=output  PseudoPeriodic=off  Frequencies=[]  VectorFormat=1-D array  Unit=A  AffineConversion=off
  ib_grid : nesl_utility/PS-Simulink Converter  PhysicalDomain=network_engine_domain  SubClassName=ps_output  LeftPortType=input  RightPortType=output  PseudoPeriodic=off  Frequencies=[]  VectorFormat=1-D array  Unit=A  AffineConversion=off
  ic_grid : nesl_utility/PS-Simulink Converter  PhysicalDomain=network_engine_domain  SubClassName=ps_output  LeftPortType=input  RightPortType=output  PseudoPeriodic=off  Frequencies=[]  VectorFormat=1-D array  Unit=A  AffineConversion=off
  ig_abc/ug_abc : Scope  NumInputPorts=2
      settings: SampleTime=param.glb_time.tc  ActiveDisplayYMinimum=-728.92703752654245  ActiveDisplayYMaximum=734.90808013997  DataLoggingVariableName=ScopeData2
  ua_grid : nesl_utility/PS-Simulink Converter  PhysicalDomain=network_engine_domain  SubClassName=ps_output  LeftPortType=input  RightPortType=output  PseudoPeriodic=off  Frequencies=[]  VectorFormat=1-D array  Unit=V  AffineConversion=off
  ub_grid : nesl_utility/PS-Simulink Converter  PhysicalDomain=network_engine_domain  SubClassName=ps_output  LeftPortType=input  RightPortType=output  PseudoPeriodic=off  Frequencies=[]  VectorFormat=1-D array  Unit=V  AffineConversion=off
  uc_grid : nesl_utility/PS-Simulink Converter  PhysicalDomain=network_engine_domain  SubClassName=ps_output  LeftPortType=input  RightPortType=output  PseudoPeriodic=off  Frequencies=[]  VectorFormat=1-D array  Unit=V  AffineConversion=off
  Ua : PMIOPort  Side=Left
  ua : PMIOPort  Port=2  Side=Right
  Ub : PMIOPort  Port=3  Side=Left
  ub : PMIOPort  Port=4  Side=Right
  Uc : PMIOPort  Port=5  Side=Left
  uc : PMIOPort  Port=6  Side=Right
  tag scope: ig_abc=global, ug_abc=global
  wires:
  Bus Creator/1 -> Selector1/1, Selector/1  "vi_data"
  Selector/1 -> [ug_abc]
  ib_grid/1 -> Bus Creator/5  "ib"
  ia_grid/1 -> Bus Creator/4  "ia"
  ic_grid/1 -> Bus Creator/6  "ic"
  ua_grid/1 -> Bus Creator/1  "ua"
  ub_grid/1 -> Bus Creator/2  "ub"
  uc_grid/1 -> Bus Creator/3  "uc"
  Selector1/1 -> [ig_abc]
  [ug_abc] -> ig_abc/ug_abc/2  "ug_abc(line)"
  [ig_abc] -> ig_abc/ug_abc/1  "ig_abc(line)"
  connections:
  Current Sensor1/LConn1 -- Ub/RConn1 -- Voltage Sensor1/LConn1
  Electrical Reference1/LConn1 -- Voltage Sensor/RConn2 -- Voltage Sensor2/RConn2 -- Voltage Sensor1/RConn2
  Voltage Sensor/RConn1 -- ua_grid/LConn1
  Current Sensor/RConn2 -- ua/RConn1
  Voltage Sensor1/RConn1 -- ub_grid/LConn1
  Voltage Sensor2/LConn1 -- Current Sensor2/LConn1 -- Uc/RConn1
  Current Sensor/LConn1 -- Ua/RConn1 -- Voltage Sensor/LConn1
  Current Sensor1/RConn2 -- ub/RConn1
  Voltage Sensor2/RConn1 -- uc_grid/LConn1
  ib_grid/LConn1 -- Current Sensor1/RConn1
  ia_grid/LConn1 -- Current Sensor/RConn1
  ic_grid/LConn1 -- Current Sensor2/RConn1
  Current Sensor2/RConn2 -- uc/RConn1

== system afe_inv_psm_n/inverter_measurement_sim/module_1 ==
  From6 : From  Commented=on  GotoTag=ileg_dc_inv_mod1
  To Workspace1 : ToWorkspace  VariableName=is_uvw_sim_mod2  SampleTime=param.glb_time.tc
      settings: MaxDataPoints=param.glb_time.Nc  Decimation=param.glb_time.decimation_tc
  To Workspace12 : ToWorkspace  Commented=on  VariableName=ileg_dc_inv_sim_mod1  SampleTime=param.glb_time.tc
      settings: MaxDataPoints=param.glb_time.Nc  Decimation=param.glb_time.decimation_tc
  To Workspace14 : ToWorkspace  VariableName=is_uvw_sim_mod1  SampleTime=param.glb_time.tc
      settings: MaxDataPoints=param.glb_time.Nc  Decimation=param.glb_time.decimation_tc
  To Workspace15 : ToWorkspace  VariableName=us_uvw_sim_mod1  SampleTime=param.glb_time.tc
      settings: MaxDataPoints=param.glb_time.Nc  Decimation=param.glb_time.decimation_tc
  To Workspace2 : ToWorkspace  VariableName=us_uvw_sim_mod2  SampleTime=param.glb_time.tc
      settings: MaxDataPoints=param.glb_time.Nc  Decimation=param.glb_time.decimation_tc
  wires:
  [us_uvw_pu_mod1] -> To Workspace15/1
  From6/1 -> To Workspace12/1
  [is_uvw_pu_mod1] -> To Workspace14/1
  [is_uvw_pu_mod2] -> To Workspace1/1
  [us_uvw_pu_mod2] -> To Workspace2/1

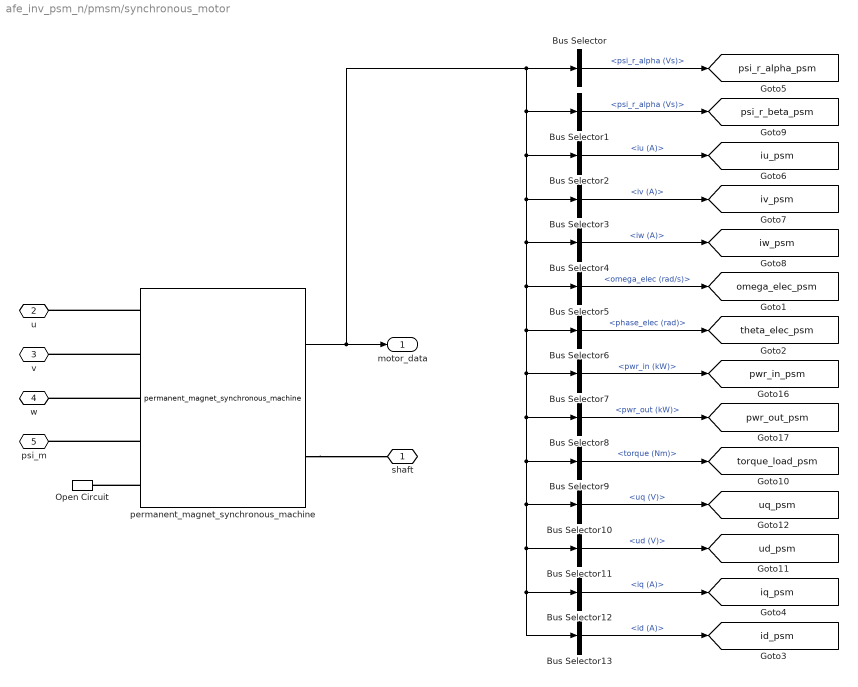
== system afe_inv_psm_n/pmsm/synchronous_motor ==
  Bus Selector : BusSelector  OutputSignals=psi_r_alpha (Vs)
  Bus Selector1 : BusSelector  OutputSignals=psi_r_alpha (Vs)
  Bus Selector10 : BusSelector  OutputSignals=uq (V)
  Bus Selector11 : BusSelector  OutputSignals=ud (V)
  Bus Selector12 : BusSelector  OutputSignals=iq (A)
  Bus Selector13 : BusSelector  OutputSignals=id (A)
  Bus Selector2 : BusSelector  OutputSignals=iu (A)
  Bus Selector3 : BusSelector  OutputSignals=iv (A)
  Bus Selector4 : BusSelector  OutputSignals=iw (A)
  Bus Selector5 : BusSelector  OutputSignals=omega_elec (rad/s)
  Bus Selector6 : BusSelector  OutputSignals=phase_elec (rad)
  Bus Selector7 : BusSelector  OutputSignals=pwr_in (kW)
  Bus Selector8 : BusSelector  OutputSignals=pwr_out (kW)
  Bus Selector9 : BusSelector  OutputSignals=torque (Nm)
  Open Circuit : fl_lib/Electrical/Electrical Elements/Open Circuit  v_specify=off  v_priority=None  v=0 V  v_nominal_specify=off  v_nominal_value=1  v_nominal_unit=V
  permanent_magnet_synchronous_machine : permanent_magnet_synchronous_machine/permanent_magnet_synchronous_machine  pp=param.psm.machine.number_poles  psi_m=param.psm.machine.psi_m  Lmu=param.psm.machine.Lmu  La=param.psm.machine.La_m/param.psm.number_of_modules  Lb=param.psm.machine.Lb_m/param.psm.number_of_modules  Rs=param.psm.machine.Rs_m/param.psm.number_of_modules  Jm=param.psm.machine.Jm_m*param.psm.number_of_modules  b_linear=param.psm.machine.load_friction_m*param.psm.number_of_modules  b_quadratic=0  h5_percent=0  h7_percent=0  psi_r_u_init=param.psm.machine.psi_m  psi_r_v_init=-param.psm.machine.psi_m/2  psi_r_w_init=-param.psm.machine.psi_m/2  omega_init=0  phase_init=0  angle_error=0
  shaft : PMIOPort  Side=Right
  u : PMIOPort  Port=2  Side=Left
  v : PMIOPort  Port=3  Side=Left
  w : PMIOPort  Port=4  Side=Left
  psi_m : PMIOPort  Port=5  Side=Left
  motor_data : Outport
  tag scope: id_psm=global, iq_psm=global, iu_psm=global, iv_psm=global, iw_psm=global, omega_elec_psm=global, psi_r_alpha_psm=global, psi_r_beta_psm=global, pwr_in_psm=global, pwr_out_psm=global, theta_elec_psm=global, torque_load_psm=global, ud_psm=global, uq_psm=global
  wires:
  permanent_magnet_synchronous_machine/1 -> Bus Selector8/1, Bus Selector10/1, Bus Selector11/1, Bus Selector12/1, Bus Selector13/1, Bus Selector9/1, Bus Selector7/1, Bus Selector6/1, Bus Selector5/1, Bus Selector4/1, Bus Selector3/1, Bus Selector2/1, Bus Selector1/1, Bus Selector/1, motor_data/1
  Bus Selector/1 -> [psi_r_alpha_psm]  "<psi_r_alpha (Vs)>"
  Bus Selector1/1 -> [psi_r_beta_psm]  "<psi_r_alpha (Vs)>"
  Bus Selector2/1 -> [iu_psm]  "<iu (A)>"
  Bus Selector3/1 -> [iv_psm]  "<iv (A)>"
  Bus Selector4/1 -> [iw_psm]  "<iw (A)>"
  Bus Selector5/1 -> [omega_elec_psm]  "<omega_elec (rad/s)>"
  Bus Selector6/1 -> [theta_elec_psm]  "<phase_elec (rad)>"
  Bus Selector7/1 -> [pwr_in_psm]  "<pwr_in (kW)>"
  Bus Selector8/1 -> [pwr_out_psm]  "<pwr_out (kW)>"
  Bus Selector9/1 -> [torque_load_psm]  "<torque (Nm)>"
  Bus Selector10/1 -> [uq_psm]  "<uq (V)>"
  Bus Selector11/1 -> [ud_psm]  "<ud (V)>"
  Bus Selector12/1 -> [iq_psm]  "<iq (A)>"
  Bus Selector13/1 -> [id_psm]  "<id (A)>"
  connections:
  permanent_magnet_synchronous_machine/RConn1 -- shaft/RConn1
  permanent_magnet_synchronous_machine/LConn1 -- u/RConn1
  permanent_magnet_synchronous_machine/LConn2 -- v/RConn1
  permanent_magnet_synchronous_machine/LConn3 -- w/RConn1
  permanent_magnet_synchronous_machine/LConn4 -- psi_m/RConn1
  permanent_magnet_synchronous_machine/LConn5 -- Open Circuit/LConn1

== system afe_inv_psm_n/scopes/grid ==
  IEC_power_meter : Scope  NumInputPorts=4
      settings: ActiveDisplayYMinimum=-139946.10544863567  ActiveDisplayYMaximum=229911.63765155774  DataLoggingVariableName=ScopeData14
  i_line_abc/u_line_abc : Scope  NumInputPorts=2
      settings: SampleTime=param.glb_time.tc  ActiveDisplayYMinimum=-2621.0463080259665  ActiveDisplayYMaximum=2989.0124297674583  DataLoggingVariableName=ScopeData20
  wires:
  [Q1p_global] -> IEC_power_meter/2  "Q1p_global"
  [Q1n_global] -> IEC_power_meter/1  "Q1n_global"
  [P1n_global] -> IEC_power_meter/4  "P1n_global"
  [P1p_global] -> IEC_power_meter/3  "P1p_global"
  [i_abc_line] -> i_line_abc/u_line_abc/1  "i_abc_line"
  [u_abc_line] -> i_line_abc/u_line_abc/2  "u_abc_line"

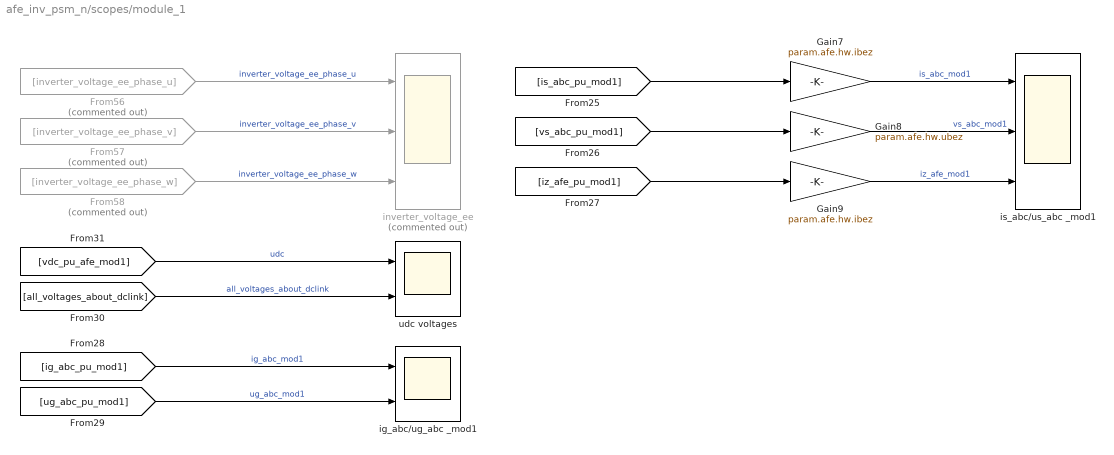
== system afe_inv_psm_n/scopes/module_1 ==
  From56 : From  Commented=on  GotoTag=inverter_voltage_ee_phase_u
  From57 : From  Commented=on  GotoTag=inverter_voltage_ee_phase_v
  From58 : From  Commented=on  GotoTag=inverter_voltage_ee_phase_w
  Gain7 : Gain  Gain=param.afe.hw.ibez
  Gain8 : Gain  Gain=param.afe.hw.ubez
  Gain9 : Gain  Gain=param.afe.hw.ibez
  ig_abc/ug_abc _mod1 : Scope  NumInputPorts=2
      settings: SampleTime=param.glb_time.tc  ActiveDisplayYMinimum=-4.4957016262667837  ActiveDisplayYMaximum=4.3239423057982735  DataLoggingVariableName=ScopeData22
  inverter_voltage_ee : Scope  Commented=on  NumInputPorts=3
      settings: SampleTime=param.glb_time.tc  ActiveDisplayYMinimum=-207.5782073641667  ActiveDisplayYMaximum=1301.7632755987056  DataLoggingVariableName=ScopeData30
  is_abc/us_abc _mod1 : Scope  NumInputPorts=3
      settings: SampleTime=param.glb_time.tc  ActiveDisplayYMinimum=-1839.9222668184293  ActiveDisplayYMaximum=1737.4961695685106  DataLoggingVariableName=ScopeData21
  udc voltages : Scope  NumInputPorts=2
      settings: SampleTime=param.glb_time.tc  ActiveDisplayYMinimum=-0.1691941690232826  ActiveDisplayYMaximum=1.5064339432334795  DataLoggingVariableName=ScopeData24
  wires:
  [ig_abc_pu_mod1] -> ig_abc/ug_abc _mod1/1  "ig_abc_mod1"
  [vdc_pu_afe_mod1] -> udc voltages/1  "udc"
  [all_voltages_about_dclink] -> udc voltages/2  "all_voltages_about_dclink"
  From58/1 -> inverter_voltage_ee/3  "inverter_voltage_ee_phase_w"
  [ug_abc_pu_mod1] -> ig_abc/ug_abc _mod1/2  "ug_abc_mod1"
  From56/1 -> inverter_voltage_ee/1  "inverter_voltage_ee_phase_u"
  From57/1 -> inverter_voltage_ee/2  "inverter_voltage_ee_phase_v"
  [iz_afe_pu_mod1] -> Gain9/1
  [vs_abc_pu_mod1] -> Gain8/1
  [is_abc_pu_mod1] -> Gain7/1
  Gain7/1 -> is_abc/us_abc _mod1/1  "is_abc_mod1"
  Gain8/1 -> is_abc/us_abc _mod1/2  "vs_abc_mod1"
  Gain9/1 -> is_abc/us_abc _mod1/3  "iz_afe_mod1"

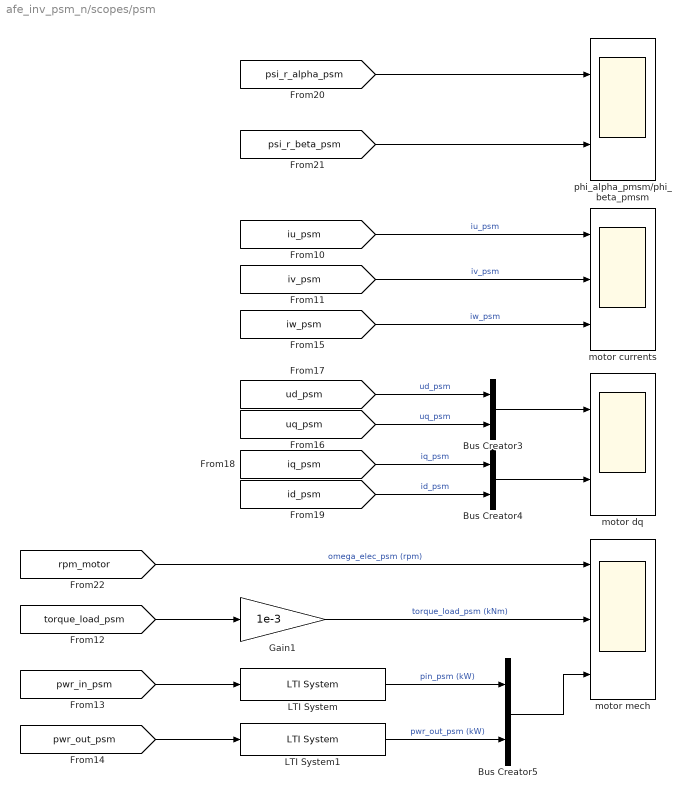
== system afe_inv_psm_n/scopes/psm ==
  Bus Creator3 : BusCreator  Inputs=2
  Bus Creator4 : BusCreator  Inputs=2
  Bus Creator5 : BusCreator  Inputs=2
  Gain1 : Gain  Gain=1e-3
  LTI System : cstblocks_lti/LTI System  sys=param.ctrl.filters.inv.SOF_50Hz.ss_c  IC=[]  PadeOrder=0
  LTI System1 : cstblocks_lti/LTI System  sys=param.ctrl.filters.inv.SOF_50Hz.ss_c  IC=[]  PadeOrder=0
  motor currents : Scope  NumInputPorts=3
      settings: SampleTime=param.glb_time.tc  ActiveDisplayYMinimum=743.22777099388588  ActiveDisplayYMaximum=952.81994596464324  DataLoggingVariableName=ScopeData17
  motor dq : Scope  NumInputPorts=2
      settings: SampleTime=param.glb_time.tc  ActiveDisplayYMinimum=-850.02239826316088  ActiveDisplayYMaximum=207.16586596148719  DataLoggingVariableName=ScopeData18
  motor mech : Scope  NumInputPorts=3
      settings: SampleTime=param.glb_time.tc  ActiveDisplayYMinimum=-2.2249642832158645  ActiveDisplayYMaximum=20.024678548942784  DataLoggingVariableName=ScopeData11
  phi_alpha_pmsm/phi_beta_pmsm : Scope  NumInputPorts=2
      settings: SampleTime=param.glb_time.tc  ActiveDisplayYMinimum=-4.8008048511588592  ActiveDisplayYMaximum=4.8008564448893649  DataLoggingVariableName=ScopeData19
  wires:
  LTI System1/1 -> Bus Creator5/2  "pwr_out_psm (kW)"
  [id_psm] -> Bus Creator4/2  "id_psm"
  [iu_psm] -> motor currents/1  "iu_psm"
  Bus Creator5/1 -> motor mech/3
  [iv_psm] -> motor currents/2  "iv_psm"
  [iq_psm] -> Bus Creator4/1  "iq_psm"
  Bus Creator4/1 -> motor dq/2
  [uq_psm] -> Bus Creator3/2  "uq_psm"
  [torque_load_psm] -> Gain1/1
  LTI System/1 -> Bus Creator5/1  "pin_psm (kW)"
  [pwr_in_psm] -> LTI System/1
  [psi_r_beta_psm] -> phi_alpha_pmsm/phi_beta_pmsm/2
  Gain1/1 -> motor mech/2  "torque_load_psm (kNm)"
  [psi_r_alpha_psm] -> phi_alpha_pmsm/phi_beta_pmsm/1
  [rpm_motor] -> motor mech/1  "omega_elec_psm (rpm)"
  [ud_psm] -> Bus Creator3/1  "ud_psm"
  [pwr_out_psm] -> LTI System1/1
  Bus Creator3/1 -> motor dq/1
  [iw_psm] -> motor currents/3  "iw_psm"
